simulink model "CCES_CHP_System"  (R2024a)
settings: Solver=ode45  StartTime=0  StopTime=86400  MaxStep=30  RelTol=1e-4
model workspace (MAT data in the model file):
  D_table = [2.05188886609 2.03582304446 2.02001391998 2.00445513561 1.98914055394 1.97406424718 1.95922048771 1.9446037392 1.93020864822 1.91603003631 1.9020628925 1.8883023662 ... (4774 elements, 77x62)]
  H_PH_vec = [168115.166404 175440.647217 182766.128031 190091.608845 197417.089659 204742.570473 212068.051287 219393.532101 226719.012915 234044.493729 241369.974543 248695.455357 ... (80 elements, 1x80)]
  H_PS_table = [474096.298336 474096.298336 474096.298336 474096.298336 474096.298336 474096.298336 474096.298336 474096.298336 474096.298336 474096.298336 474096.298336 474096.298336 ... (4960 elements, 80x62)]
  H_table = [474096.298336 475726.659021 477360.785608 478998.693717 480640.397094 482285.907734 483935.235985 485588.390649 487245.379085 488906.207299 490570.880034 492239.400856 ... (4774 elements, 77x62)]
  L_kJkg = [266.476147105 265.251949157 264.019057162 262.777320316 261.52658329 260.266686026 258.997463537 257.718745693 256.430356992 255.132116334 253.823836768 252.505325237 ... (89 elements, 1x89)]
  P_MPa = [2.41879251004 2.41979251004 2.42079251004 2.42179251004 2.42279251004 2.42379251004 2.42479251004 2.42579251004 2.42679251004 2.42779251004 2.42879251004 2.42979251004 ... (80 elements, 1x80)]
  P_PH_vec = [100000 150000 200000 250000 300000 350000 400000 450000 500000 550000 600000 650000 ... (62 elements, 1x62)]
  P_PS_vec = [100000 150000 200000 250000 300000 350000 400000 450000 500000 550000 600000 650000 ... (62 elements, 1x62)]
  P_m = [2.41879251004 2.41879251004 2.41879251004 2.41879251004 2.41879251004 2.41879251004 2.41879251004 2.41879251004 2.41879251004 2.41879251004 2.41879251004 2.41879251004 ... (80 elements, 1x80)]
  P_out = [0.0903856775851 0.0946894596647 0.0991981695679 0.103921565087 0.10886986864 0.114053789391 0.119484546432 0.125173893057 0.131134142204 0.137378193102 0.143919559183 0.150772397335 ... (100 elements, 1x100)]
  P_out_for_model = [2.41879251004 2.43293720163 2.44714230411 2.46140798189 2.47573439974 2.49012172279 2.50457011656 2.51907974695 2.53365078024 2.54828338309 2.56297772258 2.57773396617 ... (221 elements, 1x221)]
  P_sat_MPa = [2.41879251004 2.4542675608 2.49012172279 2.52635757782 2.56297772258 2.59998476905 2.63738134494 2.6751700942 2.71335367745 2.75193477255 2.79091607506 2.83030029882 ... (89 elements, 1x89)]
  P_v = [2.41879251004 2.41879251004 2.41879251004 2.41879251004 2.41879251004 2.41879251004 2.41879251004 2.41879251004 2.41879251004 2.41879251004 2.41879251004 2.41879251004 ... (100 elements, 1x100)]
  P_vec = [100000 150000 200000 250000 300000 350000 400000 450000 500000 550000 600000 650000 ... (62 elements, 1x62)]
  S_PS_vec = [865.877865734 896.930739915 927.983614097 959.036488278 990.08936246 1021.14223664 1052.19511082 1083.247985 1114.30085919 1145.35373337 1176.40660755 1207.45948173 ... (80 elements, 1x80)]
  S_table = [2625.40850187 2631.6551159 2637.86854583 2644.04935149 2650.19807314 2656.31523247 2662.40133352 2668.45686363 2674.48229423 2680.47808165 2686.44466791 2692.38248137 ... (4774 elements, 77x62)]
  T_K = [260 260.01 260.02 260.03 260.04 260.05 260.06 260.07 260.08 260.09 260.1 260.11 ... (80 elements, 1x80)]
  T_PH_table = [260 260 260 260 260 260 260 260 260 260 260 260 ... (4960 elements, 80x62)]
  T_m = [260 260 260 260 260 260 260 260 260 260 260 260 ... (80 elements, 1x80)]
  T_out = [298 298 298 298 298 298 298 298 298 298 298 298 ... (100 elements, 1x100)]
  T_out_for_model = [260 260.2 260.4 260.6 260.8 261 261.2 261.4 261.6 261.8 262 262.2 ... (221 elements, 1x221)]
  T_sat = [260 260.5 261 261.5 262 262.5 263 263.5 264 264.5 265 265.5 ... (89 elements, 1x89)]
  T_v = [260 260 260 260 260 260 260 260 260 260 260 260 ... (100 elements, 1x100)]
  T_vec = [260 262 264 266 268 270 272 274 276 278 280 282 ... (77 elements, 1x77)]
  h_f = [169441.8145 170556.967306 171675.225088 172796.648165 173921.298588 175049.240222 176180.538838 177315.262203 178453.480174 179595.264799 180740.690422 181889.833788 ... (89 elements, 1x89)]
  h_g = [435917.961605 435808.916463 435694.28225 435573.968482 435447.881878 435315.926248 435178.002376 435034.007896 434883.837166 434727.381133 434564.52719 434395.159025 ... (89 elements, 1x89)]
  m_vec = [10000 10476.1575279 10974.9876549 11497.569954 12045.0354026 12618.5688307 13219.4114847 13848.8637139 14508.287785 15199.1108295 15922.8279334 16681.005372 ... (100 elements, 1x100)]
  m_vec_for_model = [4475101.15083 4471530.78138 4467954.66783 4464372.76554 4460785.02945 4457191.41403 4453591.87327 4449986.36069 4446374.82933 4442757.23174 4439133.51996 4435503.6455 ... (221 elements, 1x221)]
  nP = 62
  nT = 77
  rho_f = [998.886219611 996.393981487 993.88678315 991.364338137 988.826352049 986.272522164 983.702537038 981.116076058 978.512808981 975.892395427 973.254484348 970.598713456 ... (89 elements, 1x89)]
  rho_g = [64.4170347985 65.4491765087 66.4967855969 67.5601486665 68.6395608905 69.7353263812 70.8477585802 71.9771806702 73.12392601 74.2883385936 75.4707735375 76.6715975945 ... (89 elements, 1x89)]
  v_vec = [0.00100111502228 0.00101024984052 0.00101946801072 0.00102877029344 0.00103815745618 0.00104763027344 0.00105718952679 0.00106683600492 0.00107657050373 0.00108639382637 0.00109630678334 0.00110631019251 ... (100 elements, 1x100)]
undefined symbols (not defined in the file or in its folder): getFluidProperty
(part 2 of 2)

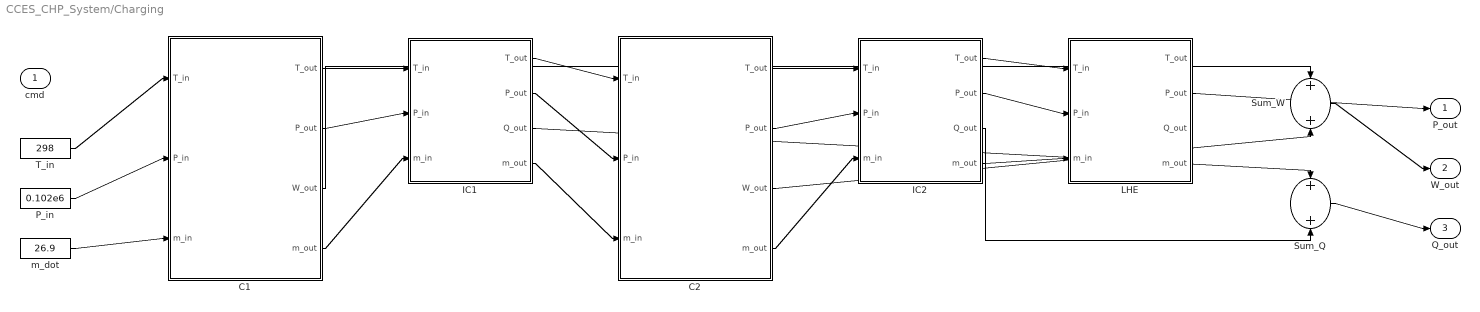
== system CCES_CHP_System/Charging ==
  cmd : Inport
  C1 : Subsystem
  C2 : Subsystem
  IC1 : Subsystem
  IC2 : Subsystem
  LHE : Subsystem
  P_in : Constant  Value=0.102e6
  Sum_Q : Sum
  Sum_W : Sum
  T_in : Constant  Value=298
  m_dot : Constant  Value=26.9
  P_out : Outport
  W_out : Outport  Port=2
  Q_out : Outport  Port=3
  wires:
  T_in/1 -> C1/1(T_in)
  P_in/1 -> C1/2(P_in)
  m_dot/1 -> C1/3(m_in)
  C1/1(T_out) -> IC1/1(T_in)
  C1/2(P_out) -> IC1/2(P_in)
  C1/4(m_out) -> IC1/3(m_in)
  IC1/1(T_out) -> C2/1(T_in)
  IC1/2(P_out) -> C2/2(P_in)
  IC1/4(m_out) -> C2/3(m_in)
  C2/1(T_out) -> IC2/1(T_in)
  C2/2(P_out) -> IC2/2(P_in)
  C2/4(m_out) -> IC2/3(m_in)
  IC2/1(T_out) -> LHE/1(T_in)
  IC2/2(P_out) -> LHE/2(P_in)
  IC2/4(m_out) -> LHE/3(m_in)
  C1/3(W_out) -> Sum_W/1
  C2/3(W_out) -> Sum_W/2
  IC1/3(Q_out) -> Sum_Q/1
  IC2/3(Q_out) -> Sum_Q/2
  LHE/2(P_out) -> P_out/1
  Sum_W/1 -> W_out/1
  Sum_Q/1 -> Q_out/1

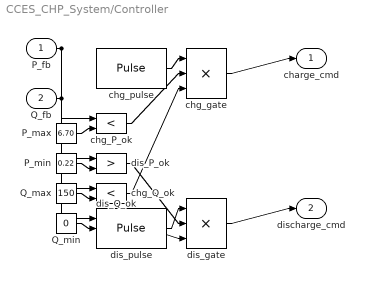
== system CCES_CHP_System/Controller ==
  P_fb : Inport
  Q_fb : Inport  Port=2
  P_max : Constant  Value=6.70
  P_min : Constant  Value=0.22
  Q_max : Constant  Value=150
  Q_min : Constant  Value=0
  chg_P_ok : RelationalOperator  Operator=<  OutDataTypeStr=boolean  RndMeth=Simplest  InputSameDT=off
  chg_Q_ok : RelationalOperator  Operator=<  OutDataTypeStr=boolean  RndMeth=Simplest  InputSameDT=off
  chg_gate : Product  Inputs=3
  chg_pulse : DiscretePulseGenerator  PulseType=Time based  Amplitude=10  Period=86400  PulseWidth=31.25
  dis_P_ok : RelationalOperator  Operator=>  OutDataTypeStr=boolean  RndMeth=Simplest  InputSameDT=off
  dis_Q_ok : RelationalOperator  Operator=>  OutDataTypeStr=boolean  RndMeth=Simplest  InputSameDT=off
  dis_gate : Product  Inputs=3
  dis_pulse : DiscretePulseGenerator  PulseType=Time based  Amplitude=10  Period=86400  PulseWidth=12.50  PhaseDelay=43200
  charge_cmd : Outport
  discharge_cmd : Outport  Port=2
  wires:
  P_fb/1 -> chg_P_ok/1, dis_P_ok/1
  P_max/1 -> chg_P_ok/2
  P_min/1 -> dis_P_ok/2
  Q_fb/1 -> chg_Q_ok/1, dis_Q_ok/1
  Q_max/1 -> chg_Q_ok/2
  Q_min/1 -> dis_Q_ok/2
  chg_pulse/1 -> chg_gate/1
  chg_P_ok/1 -> chg_gate/2
  chg_Q_ok/1 -> chg_gate/3
  chg_gate/1 -> charge_cmd/1
  dis_pulse/1 -> dis_gate/1
  dis_P_ok/1 -> dis_gate/2
  dis_Q_ok/1 -> dis_gate/3
  dis_gate/1 -> discharge_cmd/1

== system CCES_CHP_System/Discharging ==
  cmd : Inport
  T_HPT_in : Inport  Port=2
  Q_HTV_in : Inport  Port=3
  Cooler : Subsystem
  Heater : Subsystem
  P_in : Constant  Value=6.65e6
  Sum_W : Sum
  T1 : Subsystem
  T2 : Subsystem
  m_dot : Constant  Value=26.9
  W_out : Outport
  P_out : Outport  Port=2
  wires:
  Q_HTV_in/1 -> Heater/4(Q_in)
  T_HPT_in/1 -> T1/1(T_in)
  P_in/1 -> T1/2(P_in)
  m_dot/1 -> T1/3(m_in)
  T1/1(T_out) -> Heater/1(T_in)
  T1/2(P_out) -> Heater/2(P_in)
  T1/4(m_out) -> Heater/3(m_in)
  Heater/1(T_out) -> T2/1(T_in)
  Heater/2(P_out) -> T2/2(P_in)
  Heater/4(m_out) -> T2/3(m_in)
  T2/1(T_out) -> Cooler/1(T_in)
  T2/2(P_out) -> Cooler/2(P_in)
  T2/4(m_out) -> Cooler/3(m_in)
  T1/3(W_out) -> Sum_W/1
  T2/3(W_out) -> Sum_W/2
  Sum_W/1 -> W_out/1
  Cooler/2(P_out) -> P_out/1

== system CCES_CHP_System/Results ==
  W_comp : Inport
  W_turb : Inport  Port=2
  P_HPT : Inport  Port=3
  Q_HTV : Inport  Port=4
  PowerScope : Scope  NumInputPorts=2
  Q_to_MWh : Gain  Gain=1/3600
  StorageScope : Scope  NumInputPorts=2
  wires:
  W_comp/1 -> PowerScope/1
  W_turb/1 -> PowerScope/2
  Q_HTV/1 -> Q_to_MWh/1
  P_HPT/1 -> StorageScope/1
  Q_to_MWh/1 -> StorageScope/2

== system CCES_CHP_System/Storage ==
  m_dot_in : Inport
  m_dot_out : Inport  Port=2
  T_tank : Integrator  InitialCondition=298
  dTdt : Fcn  Expr=u(1)*(298-u(3))/500000 - u(2)*0.00004 + (298-u(3))/100000
  mass : Integrator  InitialCondition=383000
  mux_p : Mux  Inputs=2
  mux_t : Mux  Inputs=3
  net_m : Sum  Inputs=+-
  pressure : Fcn  Expr=u(1)*188.9*u(2)/6228/1e6
  P_MPa : Outport
  m_kg : Outport  Port=2
  T_out : Outport  Port=3
  wires:
  m_dot_in/1 -> net_m/1, mux_t/1
  m_dot_out/1 -> net_m/2, mux_t/2
  net_m/1 -> mass/1
  mass/1 -> mux_p/1, m_kg/1
  T_tank/1 -> mux_p/2, T_out/1, mux_t/3
  mux_p/1 -> pressure/1
  pressure/1 -> P_MPa/1
  mux_t/1 -> dTdt/1
  dTdt/1 -> T_tank/1

== system CCES_CHP_System/Thermal ==
  Q_in : Inport
  Q_out : Inport  Port=2
  Q_store : Integrator  InitialCondition=270000
  net_Q : Sum  Inputs=+-
  Q_MJ : Outport
  wires:
  Q_in/1 -> net_Q/1
  Q_out/1 -> net_Q/2
  net_Q/1 -> Q_store/1
  Q_store/1 -> Q_MJ/1

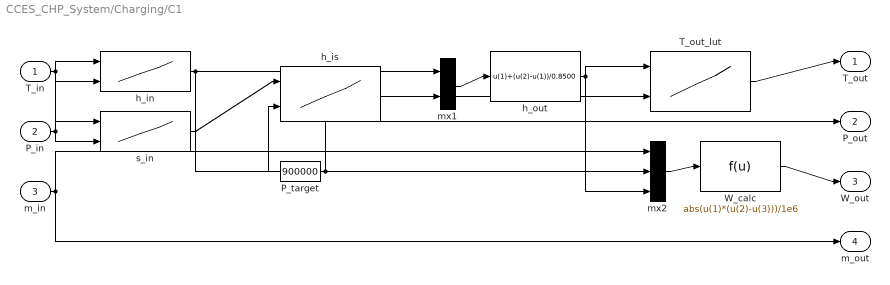
== system CCES_CHP_System/Charging/C1 ==
  T_in : Inport
  P_in : Inport  Port=2
  m_in : Inport  Port=3
  P_target : Constant  Value=900000
  T_out_lut : Lookup_n-D  BreakpointsForDimension1=H_PH_vec  BreakpointsForDimension2=P_PH_vec  Table=T_PH_table  InternalRulePriority=Speed  RndMeth=Simplest
      settings: InputPortMap=u0,u1
  W_calc : Fcn  Expr=abs(u(1)*(u(2)-u(3)))/1e6
  h_in : Lookup_n-D  BreakpointsForDimension1=T_vec  BreakpointsForDimension2=P_vec  Table=H_table  InternalRulePriority=Speed  RndMeth=Simplest
      settings: InputPortMap=u0,u1
  h_is : Lookup_n-D  BreakpointsForDimension1=S_PS_vec  BreakpointsForDimension2=P_PS_vec  Table=H_PS_table  InternalRulePriority=Speed  RndMeth=Simplest
      settings: InputPortMap=u0,u1
  h_out : Fcn  Expr=u(1)+(u(2)-u(1))/0.8500
  mx1 : Mux  Inputs=2
  mx2 : Mux  Inputs=3
  s_in : Lookup_n-D  BreakpointsForDimension1=T_vec  BreakpointsForDimension2=P_vec  Table=S_table  InternalRulePriority=Speed  RndMeth=Simplest
      settings: InputPortMap=u0,u1
  T_out : Outport
  P_out : Outport  Port=2
  W_out : Outport  Port=3
  m_out : Outport  Port=4
  wires:
  T_in/1 -> h_in/1, s_in/1
  P_in/1 -> h_in/2, s_in/2
  s_in/1 -> h_is/1
  P_target/1 -> h_is/2, T_out_lut/2, P_out/1
  h_in/1 -> mx1/1, mx2/2
  h_is/1 -> mx1/2
  mx1/1 -> h_out/1
  h_out/1 -> T_out_lut/1, mx2/3
  m_in/1 -> mx2/1, m_out/1
  mx2/1 -> W_calc/1
  T_out_lut/1 -> T_out/1
  W_calc/1 -> W_out/1

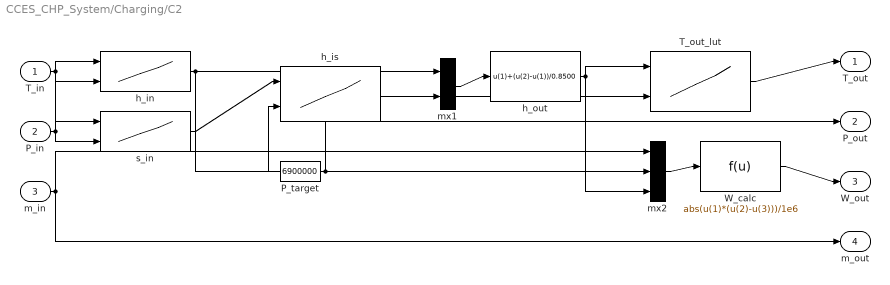
== system CCES_CHP_System/Charging/C2 ==
  T_in : Inport
  P_in : Inport  Port=2
  m_in : Inport  Port=3
  P_target : Constant  Value=6900000
  T_out_lut : Lookup_n-D  BreakpointsForDimension1=H_PH_vec  BreakpointsForDimension2=P_PH_vec  Table=T_PH_table  InternalRulePriority=Speed  RndMeth=Simplest
      settings: InputPortMap=u0,u1
  W_calc : Fcn  Expr=abs(u(1)*(u(2)-u(3)))/1e6
  h_in : Lookup_n-D  BreakpointsForDimension1=T_vec  BreakpointsForDimension2=P_vec  Table=H_table  InternalRulePriority=Speed  RndMeth=Simplest
      settings: InputPortMap=u0,u1
  h_is : Lookup_n-D  BreakpointsForDimension1=S_PS_vec  BreakpointsForDimension2=P_PS_vec  Table=H_PS_table  InternalRulePriority=Speed  RndMeth=Simplest
      settings: InputPortMap=u0,u1
  h_out : Fcn  Expr=u(1)+(u(2)-u(1))/0.8500
  mx1 : Mux  Inputs=2
  mx2 : Mux  Inputs=3
  s_in : Lookup_n-D  BreakpointsForDimension1=T_vec  BreakpointsForDimension2=P_vec  Table=S_table  InternalRulePriority=Speed  RndMeth=Simplest
      settings: InputPortMap=u0,u1
  T_out : Outport
  P_out : Outport  Port=2
  W_out : Outport  Port=3
  m_out : Outport  Port=4
  wires:
  T_in/1 -> h_in/1, s_in/1
  P_in/1 -> h_in/2, s_in/2
  s_in/1 -> h_is/1
  P_target/1 -> h_is/2, T_out_lut/2, P_out/1
  h_in/1 -> mx1/1, mx2/2
  h_is/1 -> mx1/2
  mx1/1 -> h_out/1
  h_out/1 -> T_out_lut/1, mx2/3
  m_in/1 -> mx2/1, m_out/1
  mx2/1 -> W_calc/1
  T_out_lut/1 -> T_out/1
  W_calc/1 -> W_out/1

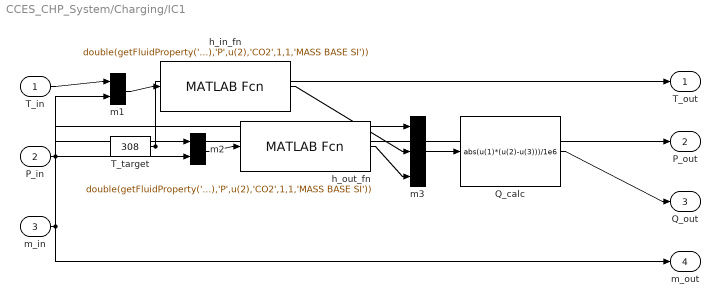
== system CCES_CHP_System/Charging/IC1 ==
  T_in : Inport
  P_in : Inport  Port=2
  m_in : Inport  Port=3
  Q_calc : Fcn  Expr=abs(u(1)*(u(2)-u(3)))/1e6
  T_target : Constant  Value=308
  h_in_fn : MATLABFcn  MATLABFcn=double(getFluidProperty('/opt/refprop/','H','T',u(1),'P',u(2),'CO2',1,1,'MASS BASE SI'))
  h_out_fn : MATLABFcn  MATLABFcn=double(getFluidProperty('/opt/refprop/','H','T',u(1),'P',u(2),'CO2',1,1,'MASS BASE SI'))
  m1 : Mux  Inputs=2
  m2 : Mux  Inputs=2
  m3 : Mux  Inputs=3
  T_out : Outport
  P_out : Outport  Port=2
  Q_out : Outport  Port=3
  m_out : Outport  Port=4
  wires:
  T_in/1 -> m1/1
  P_in/1 -> m1/2, m2/2, P_out/1
  m1/1 -> h_in_fn/1
  T_target/1 -> m2/1, T_out/1
  m2/1 -> h_out_fn/1
  m_in/1 -> m3/1, m_out/1
  h_in_fn/1 -> m3/2
  h_out_fn/1 -> m3/3
  m3/1 -> Q_calc/1
  Q_calc/1 -> Q_out/1

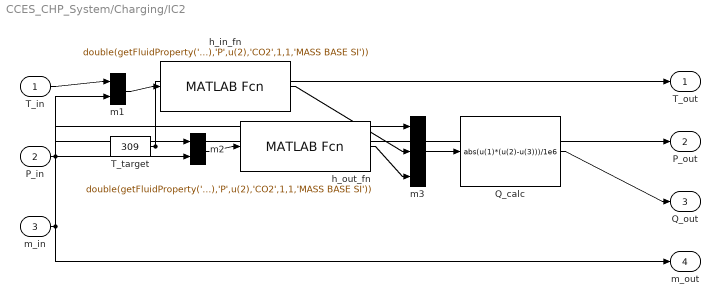
== system CCES_CHP_System/Charging/IC2 ==
  T_in : Inport
  P_in : Inport  Port=2
  m_in : Inport  Port=3
  Q_calc : Fcn  Expr=abs(u(1)*(u(2)-u(3)))/1e6
  T_target : Constant  Value=309
  h_in_fn : MATLABFcn  MATLABFcn=double(getFluidProperty('/opt/refprop/','H','T',u(1),'P',u(2),'CO2',1,1,'MASS BASE SI'))
  h_out_fn : MATLABFcn  MATLABFcn=double(getFluidProperty('/opt/refprop/','H','T',u(1),'P',u(2),'CO2',1,1,'MASS BASE SI'))
  m1 : Mux  Inputs=2
  m2 : Mux  Inputs=2
  m3 : Mux  Inputs=3
  T_out : Outport
  P_out : Outport  Port=2
  Q_out : Outport  Port=3
  m_out : Outport  Port=4
  wires:
  T_in/1 -> m1/1
  P_in/1 -> m1/2, m2/2, P_out/1
  m1/1 -> h_in_fn/1
  T_target/1 -> m2/1, T_out/1
  m2/1 -> h_out_fn/1
  m_in/1 -> m3/1, m_out/1
  h_in_fn/1 -> m3/2
  h_out_fn/1 -> m3/3
  m3/1 -> Q_calc/1
  Q_calc/1 -> Q_out/1

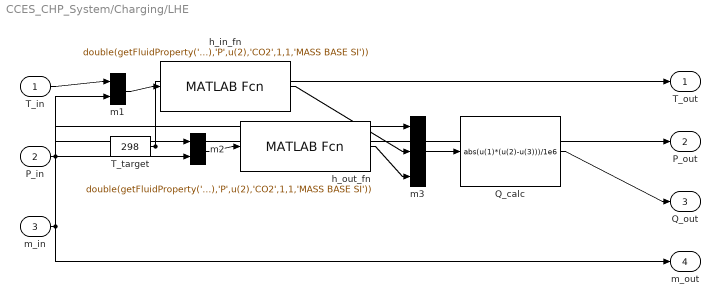
== system CCES_CHP_System/Charging/LHE ==
  T_in : Inport
  P_in : Inport  Port=2
  m_in : Inport  Port=3
  Q_calc : Fcn  Expr=abs(u(1)*(u(2)-u(3)))/1e6
  T_target : Constant  Value=298
  h_in_fn : MATLABFcn  MATLABFcn=double(getFluidProperty('/opt/refprop/','H','T',u(1),'P',u(2),'CO2',1,1,'MASS BASE SI'))
  h_out_fn : MATLABFcn  MATLABFcn=double(getFluidProperty('/opt/refprop/','H','T',u(1),'P',u(2),'CO2',1,1,'MASS BASE SI'))
  m1 : Mux  Inputs=2
  m2 : Mux  Inputs=2
  m3 : Mux  Inputs=3
  T_out : Outport
  P_out : Outport  Port=2
  Q_out : Outport  Port=3
  m_out : Outport  Port=4
  wires:
  T_in/1 -> m1/1
  P_in/1 -> m1/2, m2/2, P_out/1
  m1/1 -> h_in_fn/1
  T_target/1 -> m2/1, T_out/1
  m2/1 -> h_out_fn/1
  m_in/1 -> m3/1, m_out/1
  h_in_fn/1 -> m3/2
  h_out_fn/1 -> m3/3
  m3/1 -> Q_calc/1
  Q_calc/1 -> Q_out/1

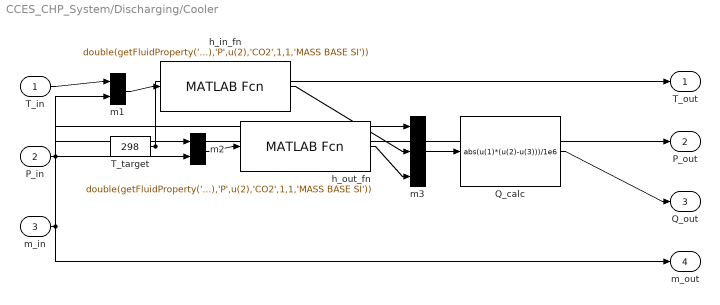
== system CCES_CHP_System/Discharging/Cooler ==
  T_in : Inport
  P_in : Inport  Port=2
  m_in : Inport  Port=3
  Q_calc : Fcn  Expr=abs(u(1)*(u(2)-u(3)))/1e6
  T_target : Constant  Value=298
  h_in_fn : MATLABFcn  MATLABFcn=double(getFluidProperty('/opt/refprop/','H','T',u(1),'P',u(2),'CO2',1,1,'MASS BASE SI'))
  h_out_fn : MATLABFcn  MATLABFcn=double(getFluidProperty('/opt/refprop/','H','T',u(1),'P',u(2),'CO2',1,1,'MASS BASE SI'))
  m1 : Mux  Inputs=2
  m2 : Mux  Inputs=2
  m3 : Mux  Inputs=3
  T_out : Outport
  P_out : Outport  Port=2
  Q_out : Outport  Port=3
  m_out : Outport  Port=4
  wires:
  T_in/1 -> m1/1
  P_in/1 -> m1/2, m2/2, P_out/1
  m1/1 -> h_in_fn/1
  T_target/1 -> m2/1, T_out/1
  m2/1 -> h_out_fn/1
  m_in/1 -> m3/1, m_out/1
  h_in_fn/1 -> m3/2
  h_out_fn/1 -> m3/3
  m3/1 -> Q_calc/1
  Q_calc/1 -> Q_out/1

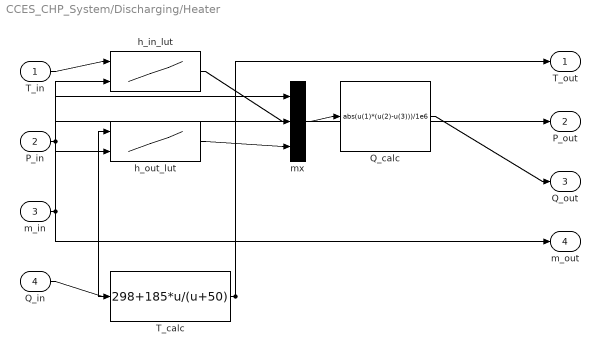
== system CCES_CHP_System/Discharging/Heater ==
  T_in : Inport
  P_in : Inport  Port=2
  m_in : Inport  Port=3
  Q_in : Inport  Port=4
  Q_calc : Fcn  Expr=abs(u(1)*(u(2)-u(3)))/1e6
  T_calc : Fcn  Expr=298+185*u/(u+50)
  h_in_lut : Lookup_n-D  BreakpointsForDimension1=T_vec  BreakpointsForDimension2=P_vec  Table=H_table  InternalRulePriority=Speed  RndMeth=Simplest
      settings: InputPortMap=u0,u1
  h_out_lut : Lookup_n-D  BreakpointsForDimension1=T_vec  BreakpointsForDimension2=P_vec  Table=H_table  InternalRulePriority=Speed  RndMeth=Simplest
      settings: InputPortMap=u0,u1
  mx : Mux  Inputs=3
  T_out : Outport
  P_out : Outport  Port=2
  Q_out : Outport  Port=3
  m_out : Outport  Port=4
  wires:
  Q_in/1 -> T_calc/1
  T_in/1 -> h_in_lut/1
  P_in/1 -> h_in_lut/2, h_out_lut/2, P_out/1
  T_calc/1 -> h_out_lut/1, T_out/1
  m_in/1 -> mx/1, m_out/1
  h_in_lut/1 -> mx/2
  h_out_lut/1 -> mx/3
  mx/1 -> Q_calc/1
  Q_calc/1 -> Q_out/1

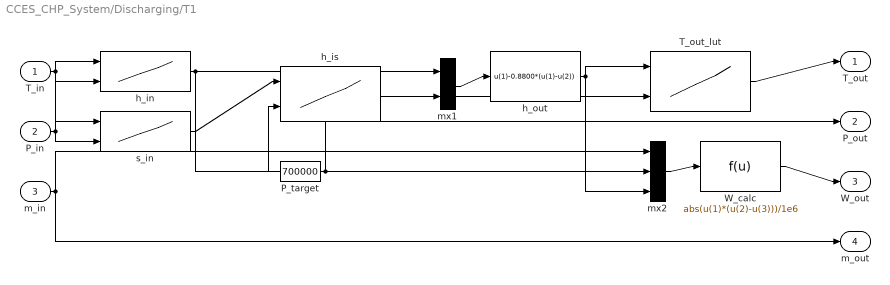
== system CCES_CHP_System/Discharging/T1 ==
  T_in : Inport
  P_in : Inport  Port=2
  m_in : Inport  Port=3
  P_target : Constant  Value=700000
  T_out_lut : Lookup_n-D  BreakpointsForDimension1=H_PH_vec  BreakpointsForDimension2=P_PH_vec  Table=T_PH_table  InternalRulePriority=Speed  RndMeth=Simplest
      settings: InputPortMap=u0,u1
  W_calc : Fcn  Expr=abs(u(1)*(u(2)-u(3)))/1e6
  h_in : Lookup_n-D  BreakpointsForDimension1=T_vec  BreakpointsForDimension2=P_vec  Table=H_table  InternalRulePriority=Speed  RndMeth=Simplest
      settings: InputPortMap=u0,u1
  h_is : Lookup_n-D  BreakpointsForDimension1=S_PS_vec  BreakpointsForDimension2=P_PS_vec  Table=H_PS_table  InternalRulePriority=Speed  RndMeth=Simplest
      settings: InputPortMap=u0,u1
  h_out : Fcn  Expr=u(1)-0.8800*(u(1)-u(2))
  mx1 : Mux  Inputs=2
  mx2 : Mux  Inputs=3
  s_in : Lookup_n-D  BreakpointsForDimension1=T_vec  BreakpointsForDimension2=P_vec  Table=S_table  InternalRulePriority=Speed  RndMeth=Simplest
      settings: InputPortMap=u0,u1
  T_out : Outport
  P_out : Outport  Port=2
  W_out : Outport  Port=3
  m_out : Outport  Port=4
  wires:
  T_in/1 -> h_in/1, s_in/1
  P_in/1 -> h_in/2, s_in/2
  s_in/1 -> h_is/1
  P_target/1 -> h_is/2, T_out_lut/2, P_out/1
  h_in/1 -> mx1/1, mx2/2
  h_is/1 -> mx1/2
  mx1/1 -> h_out/1
  h_out/1 -> T_out_lut/1, mx2/3
  m_in/1 -> mx2/1, m_out/1
  mx2/1 -> W_calc/1
  T_out_lut/1 -> T_out/1
  W_calc/1 -> W_out/1

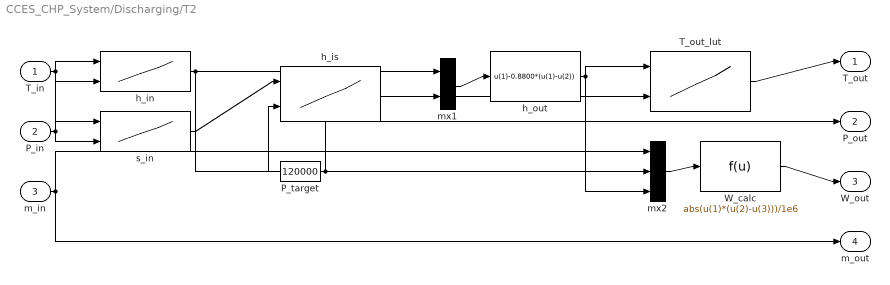
== system CCES_CHP_System/Discharging/T2 ==
  T_in : Inport
  P_in : Inport  Port=2
  m_in : Inport  Port=3
  P_target : Constant  Value=120000
  T_out_lut : Lookup_n-D  BreakpointsForDimension1=H_PH_vec  BreakpointsForDimension2=P_PH_vec  Table=T_PH_table  InternalRulePriority=Speed  RndMeth=Simplest
      settings: InputPortMap=u0,u1
  W_calc : Fcn  Expr=abs(u(1)*(u(2)-u(3)))/1e6
  h_in : Lookup_n-D  BreakpointsForDimension1=T_vec  BreakpointsForDimension2=P_vec  Table=H_table  InternalRulePriority=Speed  RndMeth=Simplest
      settings: InputPortMap=u0,u1
  h_is : Lookup_n-D  BreakpointsForDimension1=S_PS_vec  BreakpointsForDimension2=P_PS_vec  Table=H_PS_table  InternalRulePriority=Speed  RndMeth=Simplest
      settings: InputPortMap=u0,u1
  h_out : Fcn  Expr=u(1)-0.8800*(u(1)-u(2))
  mx1 : Mux  Inputs=2
  mx2 : Mux  Inputs=3
  s_in : Lookup_n-D  BreakpointsForDimension1=T_vec  BreakpointsForDimension2=P_vec  Table=S_table  InternalRulePriority=Speed  RndMeth=Simplest
      settings: InputPortMap=u0,u1
  T_out : Outport
  P_out : Outport  Port=2
  W_out : Outport  Port=3
  m_out : Outport  Port=4
  wires:
  T_in/1 -> h_in/1, s_in/1
  P_in/1 -> h_in/2, s_in/2
  s_in/1 -> h_is/1
  P_target/1 -> h_is/2, T_out_lut/2, P_out/1
  h_in/1 -> mx1/1, mx2/2
  h_is/1 -> mx1/2
  mx1/1 -> h_out/1
  h_out/1 -> T_out_lut/1, mx2/3
  m_in/1 -> mx2/1, m_out/1
  mx2/1 -> W_calc/1
  T_out_lut/1 -> T_out/1
  W_calc/1 -> W_out/1
